simulink model "single_phase_inverter"  (R2026a)
settings: Solver=ode23tb  StopTime=param.sim.simlength  FixedStep=tc  MaxStep=param.glb_time.tc
values from neighbouring files (symbols this model uses):
  param = add_template_extras(param, options)    [init_model.m]
libraries: fl_lib x45, nesl_utility x24, single_phase_transformer_lib x3, phase_shift_filter x2, phase_shift_filter_ccaller x2, three_phase_voltage_with_frt_emulator x1, power_meter_iec x1, single_phase_transformer x1, three_phase_diode_rectifier x1, three_phase_diode_rectifier_with_thermal_model x1, full_bridge_ideal_switch x1, full_bridge_mosfet_based_with_thermal_model x1
(part 4 of 4)

== system single_phase_inverter/single_phase_inverter/single phase inverter control/single_phase_inverter_ctrl/single_phase_current_control/dqpi_current_controller/i2alphabeta/first_harmonic_tracker ==
  u : Inport
  Bus Selector : BusSelector  OutputSignals=output_pu_hat,output_pu_hat_dot
  Constant1 : Constant  Value=6
  Constant2 : Constant  Value=param.glb_time.ts_inv
  Constant3 : Constant  Value=param.spinv.ctrl.omega_base
  Constant4 : Constant  Value=param.spinv.ctrl.fht_load.delta_fht
  Constant5 : Constant  Value=param.spinv.ctrl.fht_load.Ld_fht(1)
  Constant6 : Constant  Value=param.spinv.ctrl.fht_load.Ld_fht(2)
  Data Type Conversion{1..2,6..9} (6 alike) : DataTypeConversion  OutDataTypeStr=single  SaturateOnIntegerOverflow=off  RndMeth=Floor
  Data Type Conversion10 : DataTypeConversion  OutDataTypeStr=double  SaturateOnIntegerOverflow=off  RndMeth=Floor
  Data Type Conversion3 : DataTypeConversion  OutDataTypeStr=uint8  SaturateOnIntegerOverflow=off  RndMeth=Floor
  Data Type Conversion4 : DataTypeConversion  OutDataTypeStr=double  SaturateOnIntegerOverflow=off  RndMeth=Floor
  Data Type Conversion5 : DataTypeConversion  OutDataTypeStr=uint8  SaturateOnIntegerOverflow=off  RndMeth=Floor
  Gain : Gain  Gain=-1/param.afe.ctrl.fht_grid.omega_fht
  Step : Step  Time=0.0125  InitialValue=1  FinalValue=0
  first_harmonic_tracker : CCaller  FunctionName=first_harmonic_tracker_process_simulink  PortSpecificationStruct="%)30     .    B \\   8    (     @         %    \"     D    !     0         %  0 \"0    $    _    07)G3F%M90  4&]R=$YA;64 4V-O<&4     26YD97@     5'EP90      4VEZ90      27-';&]B86P   X    P    !@    @    $          4    (     0    ,    !         !   P!O=70 #@   #     &    \"     0         !0    @    !     P    $         $  # &]U=  .    .     8    (    !          %    \"     $    &     0         0  ...(+4988 chars)"
  alpha : Outport
  beta : Outport  Port=2
  wires:
  Data Type Conversion4/1 -> alpha/1
  Data Type Conversion3/1 -> first_harmonic_tracker/1
  Data Type Conversion1/1 -> first_harmonic_tracker/3
  Data Type Conversion2/1 -> first_harmonic_tracker/2
  first_harmonic_tracker/1 -> Bus Selector/1
  Bus Selector/1 -> Data Type Conversion4/1  "<output_pu_hat>"
  Step/1 -> Data Type Conversion3/1
  u/1 -> Data Type Conversion2/1
  Constant2/1 -> Data Type Conversion1/1
  Constant1/1 -> Data Type Conversion5/1
  Data Type Conversion5/1 -> first_harmonic_tracker/8
  Constant3/1 -> Data Type Conversion6/1
  Data Type Conversion6/1 -> first_harmonic_tracker/4
  Constant4/1 -> Data Type Conversion7/1
  Data Type Conversion7/1 -> first_harmonic_tracker/5
  Constant5/1 -> Data Type Conversion8/1
  Data Type Conversion8/1 -> first_harmonic_tracker/6
  Constant6/1 -> Data Type Conversion9/1
  Data Type Conversion9/1 -> first_harmonic_tracker/7
  Bus Selector/2 -> Data Type Conversion10/1  "<output_pu_hat_dot>"
  Data Type Conversion10/1 -> Gain/1
  Gain/1 -> beta/1

== system single_phase_inverter/single_phase_inverter/single phase inverter control/single_phase_inverter_ctrl/single_phase_current_control/dqpi_current_controller/i2alphabeta/phase_shift_method ==
  i_alpha : Inport
  Gain : Gain  Gain=-1
  phase shift filter : phase_shift_filter/phase shift filter  f=param.spinv.frequency_set  scaling_factor=1  ts=param.glb_time.ts_inv
  i_alpha_phase_shift_m : Outport
  i_beta_phase_shift_m : Outport  Port=2
  wires:
  i_alpha/1 -> phase shift filter/1, i_alpha_phase_shift_m/1
  Gain/1 -> i_beta_phase_shift_m/1  "i_beta_phase_shift_methos"
  phase shift filter/1 -> Gain/1

== system single_phase_inverter/single_phase_inverter/single phase inverter control/single_phase_inverter_ctrl/single_phase_current_control/dqpi_current_controller/i2alphabeta/phase_shift_method_ccaller ==
  i_alpha : Inport
  Gain : Gain  Gain=-1
  phase_shift_filter_ccaller : phase_shift_filter_ccaller/phase_shift_filter_ccaller  freq_m=param.spinv.frequency_set  ts_m=param.glb_time.ts_inv  scaling_m=1  reset_time_release=0.025  instance=0  tc_m=-1
  i_alpha_phase_shift_m : Outport
  i_beta_phase_shift_m : Outport  Port=2
  wires:
  phase_shift_filter_ccaller/1 -> Gain/1
  Gain/1 -> i_beta_phase_shift_m/1  "i_beta_phase_shift_methos"
  i_alpha/1 -> i_alpha_phase_shift_m/1, phase_shift_filter_ccaller/1

== system single_phase_inverter/single_phase_inverter/single phase inverter control/single_phase_inverter_ctrl/single_phase_current_control/dqpi_current_controller/i2alphabeta/sogi ==
  u : Inport
  Constant2 : Constant  Value=param.spinv.omega_set
  Product : Product
  Product1 : Product
  Sum1 : Sum  Inputs=|+-
  Sum3 : Sum  Inputs=-+|
  integrator_1 : Subsystem
  integrator_2 : Subsystem
  kepsilon : Gain  Gain=param.spinv.kepsilon
  ualpha : Outport
  ubeta : Outport  Port=2
  wires:
  u/1 -> ualpha/1, Sum3/2
  Sum3/1 -> kepsilon/1
  kepsilon/1 -> Sum1/1
  Sum1/1 -> Product/2
  Product/1 -> integrator_1/1(in)
  integrator_1/1(out) -> Product1/2, Sum3/1
  Constant2/1 -> Product/1, Product1/1
  Product1/1 -> integrator_2/1(in)
  integrator_2/1(out) -> ubeta/1, Sum1/2

== system single_phase_inverter/single_phase_inverter/single phase inverter control/single_phase_inverter_ctrl/single_phase_current_control/dqpi_current_controller/i2alphabeta/sogi_ccaller ==
  input : Inport
  Bus Selector : BusSelector  OutputSignals=sogi_flt_output_alpha,sogi_flt_output_beta
  CCaller : CCaller  FunctionName=sogi_flt_process_simulink  PortSpecificationStruct="%)30     .    . P   8    (     @         %    \"     <    !     0         %  0 \"0    $    _    07)G3F%M90  4&]R=$YA;64 4V-O<&4     26YD97@     5'EP90      4VEZ90      27-';&]B86P   X    P    !@    @    $          4    (     0    ,    !         !   P!O=70 #@   #     &    \"     0         !0    @    !     P    $         $  # &]U=  .    .     8    (    !          %    \"     $    &     0         0   ...(+3829 chars)"
  Constant1 : Constant  Value=param.glb_time.ts_inv
  Constant2 : Constant  Value=param.spinv.omega_set
  Constant3 : Constant  Value=param.spinv.kepsilon
  Constant4 : Constant  Value=2
  Data Type Conversion{1..2,4,6} (4 alike) : DataTypeConversion  OutDataTypeStr=single  SaturateOnIntegerOverflow=off  RndMeth=Floor
  Data Type Conversion3 : DataTypeConversion  OutDataTypeStr=uint8  SaturateOnIntegerOverflow=off  RndMeth=Floor
  Data Type Conversion5 : DataTypeConversion  OutDataTypeStr=double  SaturateOnIntegerOverflow=off  RndMeth=Floor
  Data Type Conversion7 : DataTypeConversion  OutDataTypeStr=double  SaturateOnIntegerOverflow=off  RndMeth=Floor
  Data Type Conversion8 : DataTypeConversion  OutDataTypeStr=uint8  SaturateOnIntegerOverflow=off  RndMeth=Floor
  Reset : Subsystem
  Terminator : Terminator
  Zero-Order Hold{1..6} (6 alike) : ZeroOrderHold  SampleTime=-1
  alpha : Outport
  beta : Outport  Port=2
  wires:
  Zero-Order Hold6/1 -> Data Type Conversion4/1
  Data Type Conversion4/1 -> CCaller/1
  Bus Selector/1 -> Data Type Conversion7/1  "<sogi_flt_output_alpha>"
  CCaller/1 -> Bus Selector/1
  Constant4/1 -> Zero-Order Hold5/1
  Zero-Order Hold5/1 -> Data Type Conversion3/1
  Constant2/1 -> Zero-Order Hold1/1
  Zero-Order Hold1/1 -> Data Type Conversion2/1
  Zero-Order Hold2/1 -> Data Type Conversion1/1
  Constant1/1 -> Zero-Order Hold2/1
  Reset/1(en) -> Zero-Order Hold4/1
  Zero-Order Hold4/1 -> Data Type Conversion8/1
  input/1 -> alpha/1, Zero-Order Hold6/1
  Bus Selector/2 -> Data Type Conversion5/1  "<sogi_flt_output_beta>"
  Data Type Conversion5/1 -> beta/1
  Data Type Conversion3/1 -> CCaller/6
  Data Type Conversion8/1 -> CCaller/5
  Data Type Conversion2/1 -> CCaller/3
  Data Type Conversion1/1 -> CCaller/2
  Data Type Conversion6/1 -> CCaller/4
  Zero-Order Hold3/1 -> Data Type Conversion6/1
  Constant3/1 -> Zero-Order Hold3/1
  Data Type Conversion7/1 -> Terminator/1

== system single_phase_inverter/single_phase_inverter/single phase inverter control/single_phase_inverter_ctrl/sistem_identification/open loop u//f/i2alphabeta/first_harmonic_tracker ==
  u : Inport
  Bus Selector : BusSelector  OutputSignals=output_pu_hat,output_pu_hat_dot
  Constant1 : Constant  Value=8
  Constant2 : Constant  Value=param.glb_time.ts_inv
  Constant3 : Constant  Value=param.afe.ctrl.fht_grid.omega_fht
  Constant4 : Constant  Value=param.afe.ctrl.fht_grid.delta_fht
  Constant5 : Constant  Value=param.afe.ctrl.fht_grid.Ld_fht(1)
  Constant6 : Constant  Value=param.afe.ctrl.fht_grid.Ld_fht(2)
  Data Type Conversion{1..2,6..9} (6 alike) : DataTypeConversion  OutDataTypeStr=single  SaturateOnIntegerOverflow=off  RndMeth=Floor
  Data Type Conversion10 : DataTypeConversion  OutDataTypeStr=double  SaturateOnIntegerOverflow=off  RndMeth=Floor
  Data Type Conversion3 : DataTypeConversion  OutDataTypeStr=uint8  SaturateOnIntegerOverflow=off  RndMeth=Floor
  Data Type Conversion4 : DataTypeConversion  OutDataTypeStr=double  SaturateOnIntegerOverflow=off  RndMeth=Floor
  Data Type Conversion5 : DataTypeConversion  OutDataTypeStr=uint8  SaturateOnIntegerOverflow=off  RndMeth=Floor
  Gain : Gain  Gain=-1/param.afe.ctrl.fht_grid.omega_fht
  Step : Step  Time=0.0125  InitialValue=1  FinalValue=0
  first_harmonic_tracker : CCaller  FunctionName=first_harmonic_tracker_process_simulink  PortSpecificationStruct="%)30     .    B \\   8    (     @         %    \"     D    !     0         %  0 \"0    $    _    07)G3F%M90  4&]R=$YA;64 4V-O<&4     26YD97@     5'EP90      4VEZ90      27-';&]B86P   X    P    !@    @    $          4    (     0    ,    !         !   P!O=70 #@   #     &    \"     0         !0    @    !     P    $         $  # &]U=  .    .     8    (    !          %    \"     $    &     0         0  ...(+4988 chars)"
  alpha : Outport
  beta : Outport  Port=2
  wires:
  Data Type Conversion4/1 -> alpha/1
  Data Type Conversion3/1 -> first_harmonic_tracker/1
  Data Type Conversion1/1 -> first_harmonic_tracker/3
  Data Type Conversion2/1 -> first_harmonic_tracker/2
  first_harmonic_tracker/1 -> Bus Selector/1
  Bus Selector/1 -> Data Type Conversion4/1  "<output_pu_hat>"
  Step/1 -> Data Type Conversion3/1
  u/1 -> Data Type Conversion2/1
  Constant2/1 -> Data Type Conversion1/1
  Constant1/1 -> Data Type Conversion5/1
  Data Type Conversion5/1 -> first_harmonic_tracker/8
  Constant3/1 -> Data Type Conversion6/1
  Data Type Conversion6/1 -> first_harmonic_tracker/4
  Constant4/1 -> Data Type Conversion7/1
  Data Type Conversion7/1 -> first_harmonic_tracker/5
  Constant5/1 -> Data Type Conversion8/1
  Data Type Conversion8/1 -> first_harmonic_tracker/6
  Constant6/1 -> Data Type Conversion9/1
  Data Type Conversion9/1 -> first_harmonic_tracker/7
  Bus Selector/2 -> Data Type Conversion10/1  "<output_pu_hat_dot>"
  Data Type Conversion10/1 -> Gain/1
  Gain/1 -> beta/1

== system single_phase_inverter/single_phase_inverter/single phase inverter control/single_phase_inverter_ctrl/sistem_identification/open loop u//f/i2alphabeta/phase_shift_method ==
  i_alpha : Inport
  Gain : Gain  Gain=-1
  phase shift filter : phase_shift_filter/phase shift filter  f=param.spinv.frequency_set  scaling_factor=1  ts=param.glb_time.ts_inv
  i_alpha_phase_shift_m : Outport
  i_beta_phase_shift_m : Outport  Port=2
  wires:
  i_alpha/1 -> phase shift filter/1, i_alpha_phase_shift_m/1
  Gain/1 -> i_beta_phase_shift_m/1  "i_beta_phase_shift_methos"
  phase shift filter/1 -> Gain/1

== system single_phase_inverter/single_phase_inverter/single phase inverter control/single_phase_inverter_ctrl/sistem_identification/open loop u//f/i2alphabeta/phase_shift_method_ccaller ==
  i_alpha : Inport
  Gain : Gain  Gain=-1
  phase_shift_filter_ccaller : phase_shift_filter_ccaller/phase_shift_filter_ccaller  freq_m=param.spinv.frequency_set  ts_m=param.glb_time.ts_inv  scaling_m=1  reset_time_release=0.025  instance=2  tc_m=-1
  i_alpha_phase_shift_m : Outport
  i_beta_phase_shift_m : Outport  Port=2
  wires:
  phase_shift_filter_ccaller/1 -> Gain/1
  Gain/1 -> i_beta_phase_shift_m/1  "i_beta_phase_shift_methos"
  i_alpha/1 -> i_alpha_phase_shift_m/1, phase_shift_filter_ccaller/1

== system single_phase_inverter/single_phase_inverter/single phase inverter control/single_phase_inverter_ctrl/sistem_identification/open loop u//f/i2alphabeta/sogi ==
  u : Inport
  Constant2 : Constant  Value=param.spinv.omega_set
  Product : Product
  Product1 : Product
  Sum1 : Sum  Inputs=|+-
  Sum3 : Sum  Inputs=-+|
  integrator_1 : Subsystem
  integrator_2 : Subsystem
  kepsilon : Gain  Gain=param.spinv.kepsilon
  ualpha : Outport
  ubeta : Outport  Port=2
  wires:
  u/1 -> ualpha/1, Sum3/2
  Sum3/1 -> kepsilon/1
  kepsilon/1 -> Sum1/1
  Sum1/1 -> Product/2
  Product/1 -> integrator_1/1(in)
  integrator_1/1(out) -> Product1/2, Sum3/1
  Constant2/1 -> Product/1, Product1/1
  Product1/1 -> integrator_2/1(in)
  integrator_2/1(out) -> ubeta/1, Sum1/2

== system single_phase_inverter/single_phase_inverter/single phase inverter control/single_phase_inverter_ctrl/sistem_identification/open loop u//f/i2alphabeta/sogi_ccaller ==
  input : Inport
  Bus Selector : BusSelector  OutputSignals=sogi_flt_output_alpha,sogi_flt_output_beta
  CCaller : CCaller  FunctionName=sogi_flt_process_simulink  PortSpecificationStruct="%)30     .    . P   8    (     @         %    \"     <    !     0         %  0 \"0    $    _    07)G3F%M90  4&]R=$YA;64 4V-O<&4     26YD97@     5'EP90      4VEZ90      27-';&]B86P   X    P    !@    @    $          4    (     0    ,    !         !   P!O=70 #@   #     &    \"     0         !0    @    !     P    $         $  # &]U=  .    .     8    (    !          %    \"     $    &     0         0   ...(+3829 chars)"
  Constant1 : Constant  Value=param.glb_time.ts_inv
  Constant2 : Constant  Value=param.spinv.omega_set
  Constant3 : Constant  Value=param.spinv.kepsilon
  Constant4 : Constant  Value=4
  Data Type Conversion{1..2,4,6} (4 alike) : DataTypeConversion  OutDataTypeStr=single  SaturateOnIntegerOverflow=off  RndMeth=Floor
  Data Type Conversion3 : DataTypeConversion  OutDataTypeStr=uint8  SaturateOnIntegerOverflow=off  RndMeth=Floor
  Data Type Conversion5 : DataTypeConversion  OutDataTypeStr=double  SaturateOnIntegerOverflow=off  RndMeth=Floor
  Data Type Conversion7 : DataTypeConversion  OutDataTypeStr=double  SaturateOnIntegerOverflow=off  RndMeth=Floor
  Data Type Conversion8 : DataTypeConversion  OutDataTypeStr=uint8  SaturateOnIntegerOverflow=off  RndMeth=Floor
  Reset : Subsystem
  Terminator : Terminator
  Zero-Order Hold{1..6} (6 alike) : ZeroOrderHold  SampleTime=-1
  alpha : Outport
  beta : Outport  Port=2
  wires:
  Zero-Order Hold6/1 -> Data Type Conversion4/1
  Data Type Conversion4/1 -> CCaller/1
  Bus Selector/1 -> Data Type Conversion7/1  "<sogi_flt_output_alpha>"
  CCaller/1 -> Bus Selector/1
  Constant4/1 -> Zero-Order Hold5/1
  Zero-Order Hold5/1 -> Data Type Conversion3/1
  Constant2/1 -> Zero-Order Hold1/1
  Zero-Order Hold1/1 -> Data Type Conversion2/1
  Zero-Order Hold2/1 -> Data Type Conversion1/1
  Constant1/1 -> Zero-Order Hold2/1
  Reset/1(en) -> Zero-Order Hold4/1
  Zero-Order Hold4/1 -> Data Type Conversion8/1
  input/1 -> alpha/1, Zero-Order Hold6/1
  Bus Selector/2 -> Data Type Conversion5/1  "<sogi_flt_output_beta>"
  Data Type Conversion5/1 -> beta/1
  Data Type Conversion3/1 -> CCaller/6
  Data Type Conversion8/1 -> CCaller/5
  Data Type Conversion2/1 -> CCaller/3
  Data Type Conversion1/1 -> CCaller/2
  Data Type Conversion6/1 -> CCaller/4
  Zero-Order Hold3/1 -> Data Type Conversion6/1
  Constant3/1 -> Zero-Order Hold3/1
  Data Type Conversion7/1 -> Terminator/1

== system single_phase_inverter/single_phase_inverter/single phase inverter control/single_phase_inverter_ctrl/single_phase_current_control/dqpi_current_controller/i2alphabeta/sogi/integrator_1 ==
  in : Inport
  Sum : Sum  Inputs=|++
  sample_time : Gain  Gain=param.glb_time.ts_inv
  unit_delay_1 : UnitDelay  SampleTime=-1
  out : Outport
  wires:
  in/1 -> sample_time/1
  sample_time/1 -> Sum/1
  Sum/1 -> unit_delay_1/1, out/1
  unit_delay_1/1 -> Sum/2

== system single_phase_inverter/single_phase_inverter/single phase inverter control/single_phase_inverter_ctrl/single_phase_current_control/dqpi_current_controller/i2alphabeta/sogi/integrator_2 ==
  in : Inport
  Sum : Sum  Inputs=|++
  sample_time : Gain  Gain=param.glb_time.ts_inv
  unit_delay_1 : UnitDelay  SampleTime=-1
  out : Outport
  wires:
  sample_time/1 -> Sum/1
  in/1 -> sample_time/1
  Sum/1 -> out/1, unit_delay_1/1
  unit_delay_1/1 -> Sum/2

== system single_phase_inverter/single_phase_inverter/single phase inverter control/single_phase_inverter_ctrl/single_phase_current_control/dqpi_current_controller/i2alphabeta/sogi_ccaller/Reset ==
  Step : Step  Time=0.025  InitialValue=1  FinalValue=0
  en : Outport
  wires:
  Step/1 -> en/1

== system single_phase_inverter/single_phase_inverter/single phase inverter control/single_phase_inverter_ctrl/sistem_identification/open loop u//f/i2alphabeta/sogi/integrator_1 ==
  in : Inport
  Sum : Sum  Inputs=|++
  sample_time : Gain  Gain=param.glb_time.ts_inv
  unit_delay_1 : UnitDelay  SampleTime=-1
  out : Outport
  wires:
  in/1 -> sample_time/1
  sample_time/1 -> Sum/1
  Sum/1 -> unit_delay_1/1, out/1
  unit_delay_1/1 -> Sum/2

== system single_phase_inverter/single_phase_inverter/single phase inverter control/single_phase_inverter_ctrl/sistem_identification/open loop u//f/i2alphabeta/sogi/integrator_2 ==
  in : Inport
  Sum : Sum  Inputs=|++
  sample_time : Gain  Gain=param.glb_time.ts_inv
  unit_delay_1 : UnitDelay  SampleTime=-1
  out : Outport
  wires:
  sample_time/1 -> Sum/1
  in/1 -> sample_time/1
  Sum/1 -> out/1, unit_delay_1/1
  unit_delay_1/1 -> Sum/2

== system single_phase_inverter/single_phase_inverter/single phase inverter control/single_phase_inverter_ctrl/sistem_identification/open loop u//f/i2alphabeta/sogi_ccaller/Reset ==
  Step : Step  Time=0.025  InitialValue=1  FinalValue=0
  en : Outport
  wires:
  Step/1 -> en/1

== matlab function single_phase_inverter/single phase inverter control/single_phase_inverter_ctrl/impedance_measure/Subsystem/MATLAB Function ==
  data: u input; y output; Vdc_FS input; Vac_FS input; Xbez input
function y = scaling(u, Vdc_FS, Vac_FS, Xbez)

y = Vdc_FS/Vac_FS*Xbez * u;

== matlab function single_phase_inverter/single phase inverter control/single_phase_inverter_ctrl/sistem_identification/open loop u//f/dq2alphabeta/MATLAB Function ==
  data: d input; alpha output; q input; phase input; beta output
function [alpha, beta] = dq2alphabeta(d, q, phase)

alpha = d*cos(phase) - q*sin(phase);
beta = d*sin(phase) + q*cos(phase);

== matlab function single_phase_inverter/single phase inverter control/single_phase_inverter_ctrl/single_phase_current_control/dqpi_current_controller/alphabeta2dq/MATLAB Function ==
  data: alpha input; d output; beta input; phase input; q output
function [d, q] = alphabeta2dq(alpha, beta, phase)

d = alpha*cos(phase) + beta*sin(phase);
q = -alpha*sin(phase) + beta*cos(phase);

== matlab function single_phase_inverter/single phase inverter control/single_phase_inverter_ctrl/single_phase_current_control/dqpi_current_controller/dq2alphabeta/MATLAB Function ==
  data: d input; alpha output; q input; phase input; beta output
function [alpha, beta] = dq2alphabeta(d, q, phase)

alpha = d*cos(phase) - q*sin(phase);
beta = d*sin(phase) + q*cos(phase);

== matlab function single_phase_inverter/single phase inverter control/single_phase_inverter_ctrl/phase generator/bounder1 ==
  data: u input; y output
function y = bounder(u)
    
    y = -pi + mod(u+3*pi,2*pi);
   
end
